simulink model "Vehicle1D_Component_harness_model"  (R2023a)
settings: Solver=daessc  StartTime=0.0  StopTime=100  RelTol=1e-3  AbsTol=1e-3
PreLoadFcn:
  | Vehicle1D_Component_harness_setup
libraries: fl_lib x3, nesl_utility x2
settings Model: Creator=isaacito  LastModifiedBy=isaacito
settings SolverCC: AutoScaleAbsTol=off  AlgebraicLoopSolver=TrustRegion
settings DataIOCC: DSMLogging=off
settings OptimizationCC: ReuseModelBlockBuffer=off
settings DebuggingCC: UnconnectedInputMsg=warning  UnconnectedOutputMsg=warning  UnconnectedLineMsg=warning
settings ModelReferenceCC: EnableRefExpFcnMdlSchedulingChecks=on
settings RTWCC: DLArmComputeVersion=19.05
settings SimscapeCC: SimscapeLogType=all  SimscapeLogSimulationStatistics=on  SimscapeLogLimitData=off

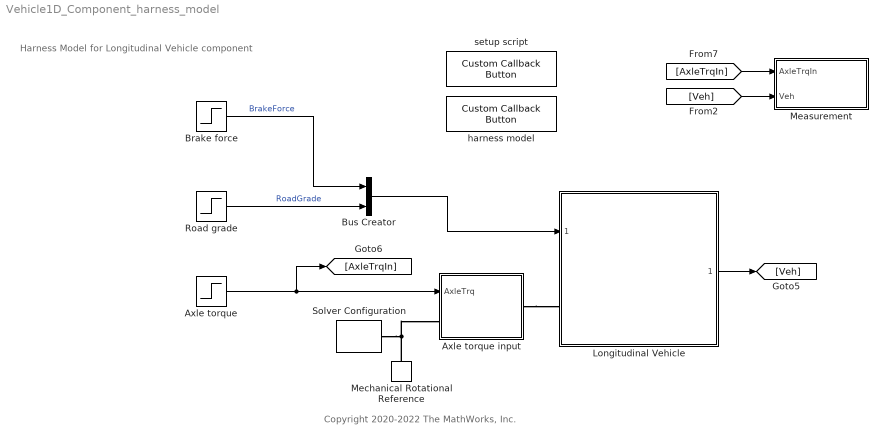
== system Vehicle1D_Component_harness_model ==
  note: Harness Model for Longitudinal Vehicle component
  note: Copyright 2020-2022 The MathWorks, Inc.
  Axle torque : Step  Time=20  Before=500  After=0  SampleTime=0
      settings: AttributesFormatString=|
      | Step time: %<Time>
      | Initial: %<Before>
      | Final: %<After>
  Axle torque input : Subsystem
  Brake force : Step  Time=70  After=500  SampleTime=0
      settings: AttributesFormatString=|
      | Step time: %<Time>
      | Initial: %<Before>
      | Final: %<After>
  Bus Creator : BusCreator  Inputs=2
  Longitudinal Vehicle : Subsystem  ReferencedSubsystem=Vehicle1D_refsub_Basic
  Measurement : Subsystem
  Mechanical Rotational Reference : fl_lib/Mechanical/Rotational Elements/Mechanical Rotational Reference
  Road grade : Step  Time=50  Before=-5  After=0  SampleTime=0
      settings: AttributesFormatString=|
      | Step time: %<Time>
      | Initial: %<Before>
      | Final: %<After>
  Solver Configuration : nesl_utility/Solver Configuration  PhysicalDomain=network_engine_domain  SubClassName=solver  LeftPortType=input  RightPortType=generic  Tones=[]  Harmonics=[]  SimulateNoise=off  Profile=off  UseLocalSampling=off  EnableSwitchedLinearOptims=on  FrequencyDomain=off  UseCCode=off  RelTol=0.001  AbsTol=1e-06  MinStep=1e-09  ToWorkspace=off  RevertToSquareIcSolve=off  NumHomotopyIterations=100  PhasorMode=off  PhasorModeNumHarmonics=1  ConsistencySolver=NEWTON_FTOL  IndexReductionMethod=DerivativeReplacement  DoDC=off  ResidualTolerance=1e-09  ConsistencyTolSource=GLOBAL  ConsistencyAbsTol=0.001  ConsistencyRelTol=0.001  ConsistencyTolFactor=0.001  UseLocalSolver=off  LocalSolverChoice=NE_BACKWARD_EULER_ADVANCER  ResolveIndetEquations=on  FunctionEvalNumThread=1  LocalSolverSampleTime=0.001  DoFixedCost=off  MaxNonlinIter=3  MaxModeIter=2  ComputeImpulses=off  ImpulseIterations=2  LinearAlgebra=auto  LinearAlgebraNumThread=0  EquationFormulation=NE_TIME_EF  DelaysMemoryBudget=1024  AutomaticFiltering=on  FilteringTimeConstant=0.001  PartitionStorageMethod=AS_NEEDED  PartitionMemoryBudget=1024  PartitionMethod=ROBUST
      settings: AttributesFormatString=Local solver %<UseLocalSolver>
  harness model : CustomCallbackButton  Configuration="{\"components\":[{\"name\":\"BackgroundImageComponent\",\"settings\":{\"image\":{\"size\":[0,0],\"src\":\"default\",\"srcOrientation\":\"Right\"},\"position\":[0,0,1,1]}},{\"name\":\"ButtonStateComponent\",\"settings\":{\"buttonType\":\"momentary\",\"clickFcn\":\"Vehicle1D_Component_resetHarnessModel\\n\",\"onValue\":1,\"position\":[0,0,1,1],\"pressDelay\":\"500\",\"pressFcn\":\"\",\"repeatInterval\":\"0\",\"states\":[{\"horizontalAlignment\":\"center\",\"image\":{\"position\":[0,0,1,1],\"src\":\"default\",\"srcOrientation\":\"Right\"},\"label\":{\"color\":[0.01176470588,0.01176470588,0.01176470588,1],\"icon\":{\"size\":[0,0],\"src\":\"default\",\"srcOrientation\":\"Right\"},\"iconPlacement\":\"left\",\"text\":{\"content\":\"Reset\"}},\"labelOffset\":[0,0],\"verticalAlignment\":\"middle\"},{\"horizontalAlignment\":\"center\",\"image\":{\"position\":[0,0,1,1],\"src\":\"default\",\"srcOrientation\":\"Right\"},\"label\":{\"color\":[0.01176470588,0.01176470588,0.01176470588,1],\"icon\":{\"size\":[0,0],\"src\":\"default\",\"srcOrientation\":\"Right\"},\"iconPlacement\":\"left\",\"text\":{\"content\":\"Reset\"}},\"labelOffset\":[0,0],\"verticalAlignment\":\"middle\"},{\"horizontalAlignment\":\"center\",\"image\":{\"position\":[0,0,1,1],\"src\":\"default\",\"srcOrientation\":\"Right\"},\"label\":{\"color\":[0.01176470588,0.01176470588,0.01176470588,1],\"icon\":{\"size\":[0,0],\"src\":\"default\",\"srcOrientation\":\"Right\"},\"iconPlacement\":\"left\",\"text\":{\"content\":\"Reset\"}},\"labelOffset\":[0,0],\"verticalAlignment\":\"middle\"},{\"horizontalAlignment\":\"center\",\"image\":{\"position\":[0,0,1,1],\"src\":\"default\",\"srcOrientation\":\"Right\"},\"label\":{\"color\":[0.01176470588,0.01176470588,0.01176470588,1],\"icon\":{\"size\":[0,0],\"src\":\"default\",\"srcOrientation\":\"Right\"},\"iconPlacement\":\"left\",\"text\":{\"content\":\"Reset\"}},\"labelOffset\":[0,0],\"verticalAlignment\":\"middle\"}]}},{\"name\":\"ForegroundImageComponent\",\"settings\":{\"image\":{\"size\":[0,0],\"src\":\"default\",\"srcOrientation\":\"Right\"},\"isForeground\":1,\"position\":[0,0,1,1]}}],\"settings\":{\"BindingType\":\"standalone\",\"backgroundColor\":[244,244,244,1],\"backgroundOffset\":0.2,\"backgroundOpacity\":1,\"fixedAspectRatio\":\"off\",\"foregroundColor\":[0.01176470588,0.01176470588,0.01176470588,1],\"migratedFromLegacy\":true,\"useBackgroundColor\":true,\"variant\":\"callback\",\"version\":\"R2023a\"},\"type\":\"Button\"}"  CustomBackgroundColor="{\"color\":[0.9568627451,0.9568627451,0.9568627451],\"show\":true}"
  setup script : CustomCallbackButton  Configuration="{\"components\":[{\"name\":\"BackgroundImageComponent\",\"settings\":{\"image\":{\"size\":[0,0],\"src\":\"default\",\"srcOrientation\":\"Right\"},\"position\":[0,0,1,1]}},{\"name\":\"ButtonStateComponent\",\"settings\":{\"buttonType\":\"momentary\",\"clickFcn\":\"edit Vehicle1D_Component_harness_setup\\n\",\"onValue\":1,\"position\":[0,0,1,1],\"pressDelay\":\"500\",\"pressFcn\":\"\",\"repeatInterval\":\"0\",\"states\":[{\"horizontalAlignment\":\"center\",\"image\":{\"position\":[0,0,1,1],\"src\":\"default\",\"srcOrientation\":\"Right\"},\"label\":{\"color\":[0.01176470588,0.01176470588,0.01176470588,1],\"icon\":{\"size\":[0,0],\"src\":\"default\",\"srcOrientation\":\"Right\"},\"iconPlacement\":\"left\",\"text\":{\"content\":\"Open\"}},\"labelOffset\":[0,0],\"verticalAlignment\":\"middle\"},{\"horizontalAlignment\":\"center\",\"image\":{\"position\":[0,0,1,1],\"src\":\"default\",\"srcOrientation\":\"Right\"},\"label\":{\"color\":[0.01176470588,0.01176470588,0.01176470588,1],\"icon\":{\"size\":[0,0],\"src\":\"default\",\"srcOrientation\":\"Right\"},\"iconPlacement\":\"left\",\"text\":{\"content\":\"Open\"}},\"labelOffset\":[0,0],\"verticalAlignment\":\"middle\"},{\"horizontalAlignment\":\"center\",\"image\":{\"position\":[0,0,1,1],\"src\":\"default\",\"srcOrientation\":\"Right\"},\"label\":{\"color\":[0.01176470588,0.01176470588,0.01176470588,1],\"icon\":{\"size\":[0,0],\"src\":\"default\",\"srcOrientation\":\"Right\"},\"iconPlacement\":\"left\",\"text\":{\"content\":\"Open\"}},\"labelOffset\":[0,0],\"verticalAlignment\":\"middle\"},{\"horizontalAlignment\":\"center\",\"image\":{\"position\":[0,0,1,1],\"src\":\"default\",\"srcOrientation\":\"Right\"},\"label\":{\"color\":[0.01176470588,0.01176470588,0.01176470588,1],\"icon\":{\"size\":[0,0],\"src\":\"default\",\"srcOrientation\":\"Right\"},\"iconPlacement\":\"left\",\"text\":{\"content\":\"Open\"}},\"labelOffset\":[0,0],\"verticalAlignment\":\"middle\"}]}},{\"name\":\"ForegroundImageComponent\",\"settings\":{\"image\":{\"size\":[0,0],\"src\":\"default\",\"srcOrientation\":\"Right\"},\"isForeground\":1,\"position\":[0,0,1,1]}}],\"settings\":{\"BindingType\":\"standalone\",\"backgroundColor\":[244,244,244,1],\"backgroundOffset\":0.2,\"backgroundOpacity\":1,\"fixedAspectRatio\":\"off\",\"foregroundColor\":[0.01176470588,0.01176470588,0.01176470588,1],\"migratedFromLegacy\":true,\"useBackgroundColor\":true,\"variant\":\"callback\",\"version\":\"R2023a\"},\"type\":\"Button\"}"  CustomBackgroundColor="{\"color\":[0.9568627451,0.9568627451,0.9568627451],\"show\":true}"
  wires:
  [Veh] -> Measurement/2(Veh)
  [AxleTrqIn] -> Measurement/1(AxleTrqIn)
  Bus Creator/1 -> Longitudinal Vehicle/1
  Road grade/1 -> Bus Creator/2  "RoadGrade"
  Brake force/1 -> Bus Creator/1  "BrakeForce"
  Axle torque/1 -> [AxleTrqIn], Axle torque input/1(AxleTrq)
  Longitudinal Vehicle/1 -> [Veh]
  connections:
  Axle torque input/RConn1 -- Longitudinal Vehicle/LConn1
  Mechanical Rotational Reference/LConn1 -- Solver Configuration/RConn1 -- Axle torque input/LConn1

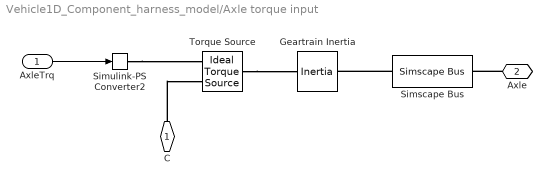
== system Vehicle1D_Component_harness_model/Axle torque input ==
  AxleTrq : Inport
  Geartrain Inertia : fl_lib/Mechanical/Rotational Elements/Inertia  inertia=10*0.1^2 kg*m^2  num_ports=foundation.enum.numPorts2.two  w_specify=on  w_priority=None  w=0 rpm  w_nominal_specify=off  w_nominal_unit=rad/s  w_nominal_value=1  t_specify=off  t_priority=None  t=0 N*m  t_nominal_specify=off  t_nominal_unit=N*m  t_nominal_value=1
      settings: InternalSimscapePortConfiguration="{\"Bottom\":[],\"Left\":[{\"id\":\"I\",\"label\":\"\",\"type\":\"foundation.mechanical.rotational.rotational\"}],\"Right\":[{\"id\":\"J\",\"label\":\"\",\"type\":\"foundation.mechanical.rotational.rotational\"}],\"Top\":[]}"
      settings: AttributesFormatString=|
      | %<inertia>
      | %<inertia_unit>
  Simscape Bus : SimscapeBus  HierarchyStrings=AngSpd  ConnectionType=Bus: Bus_Rotational
      settings: AttributesFormatString=%<ConnectionType>
  Simulink-PS Converter2 : nesl_utility/Simulink-PS Converter  PhysicalDomain=network_engine_domain  SubClassName=ps_input  LeftPortType=input  RightPortType=output  PseudoPeriodic=off  Frequencies=[]  NoiseDistribution=none  NoiseParameters=[]  Unit=N*m  AffineConversion=off  FilteringAndDerivatives=filter  SimscapeFilterOrder=1  InputFilterTimeConstant=0.001  UdotUserProvided=0
  Torque Source : fl_lib/Mechanical/Mechanical Sources/Ideal Torque Source
  C : PMIOPort  Side=Left
  Axle : PMIOPort  Port=2  Side=Right
  wires:
  AxleTrq/1 -> Simulink-PS Converter2/1
  connections:
  C/RConn1 -- Torque Source/RConn2
  Simulink-PS Converter2/RConn1 -- Torque Source/RConn1
  Torque Source/LConn1 -- Geartrain Inertia/RConn1
  Simscape Bus/LConn1 -- Geartrain Inertia/LConn1
  Axle/RConn1 -- Simscape Bus/RConn1

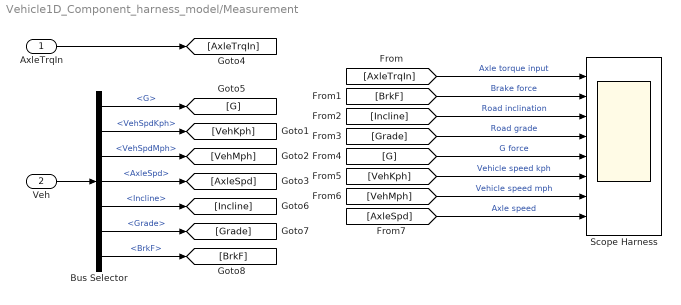
== system Vehicle1D_Component_harness_model/Measurement ==
  AxleTrqIn : Inport
  Veh : Inport  Port=2
  Bus Selector : BusSelector  OutputSignals=G,VehSpdKph,VehSpdMph,AxleSpd,Incline,Grade,BrkF
  Scope Harness : Scope  NumInputPorts=8
  wires:
  Veh/1 -> Bus Selector/1
  AxleTrqIn/1 -> [AxleTrqIn]
  Bus Selector/1 -> [G]  "<G>"
  Bus Selector/2 -> [VehKph]  "<VehSpdKph>"
  Bus Selector/3 -> [VehMph]  "<VehSpdMph>"
  Bus Selector/4 -> [AxleSpd]  "<AxleSpd>"
  Bus Selector/5 -> [Incline]  "<Incline>"
  Bus Selector/6 -> [Grade]  "<Grade>"
  Bus Selector/7 -> [BrkF]  "<BrkF>"
  [Grade] -> Scope Harness/4  "Road grade"
  [Incline] -> Scope Harness/3  "Road inclination"
  [G] -> Scope Harness/5  "G force"
  [BrkF] -> Scope Harness/2  "Brake force"
  [VehKph] -> Scope Harness/6  "Vehicle speed kph"
  [AxleTrqIn] -> Scope Harness/1  "Axle torque input"
  [VehMph] -> Scope Harness/7  "Vehicle speed mph"
  [AxleSpd] -> Scope Harness/8  "Axle speed"
